simulink model "week8_heading_control"  (R2026a)
settings: Solver=VariableStepAuto
values from neighbouring files (symbols this model uses):
  alpha = (1 - sind(phi_lead))/(1 + sind(phi_lead))    [Week8.m]
  B = 0.15    [Week8.m]
  D = 3.2e-7    (= 3.2e-07)    [Week8.m]
  gear = 9.6    [Week8.m]
  J_new = 5.4836e-6    (= 5.4836e-06)    [Week8.m]
  Kb = 0.009    [Week8.m]
  Kp_P = 0.05    [Week8.m]
  Kph = sqrt(alpha)/mag(k_wc)    [Week8.m]
  Kt = 0.009    [Week8.m]
  L = 0.01    [Week8.m]
  R = 6.8    [Week8.m]
  taud = 1/(wc_lead*sqrt(alpha))    [Week8.m]
  Ts = 0.001    [Week8.m]
  useZOH = 1    [Week8.m]
  wrad = 0.0315    [Week8.m]
libraries: simulink x1
settings Model: Creator=sophiewinther  LastModifiedBy=sahra

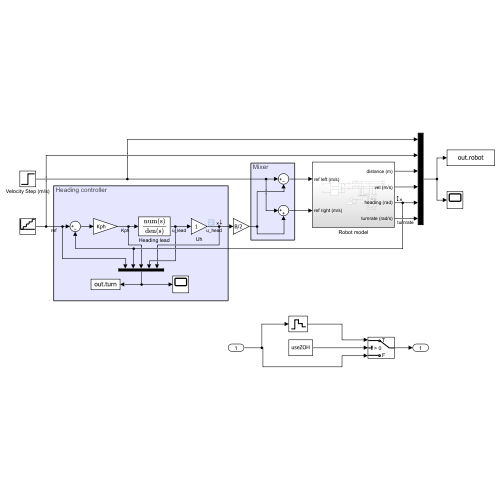
[thumbnail: Simulink's stored preview of the top-level diagram]
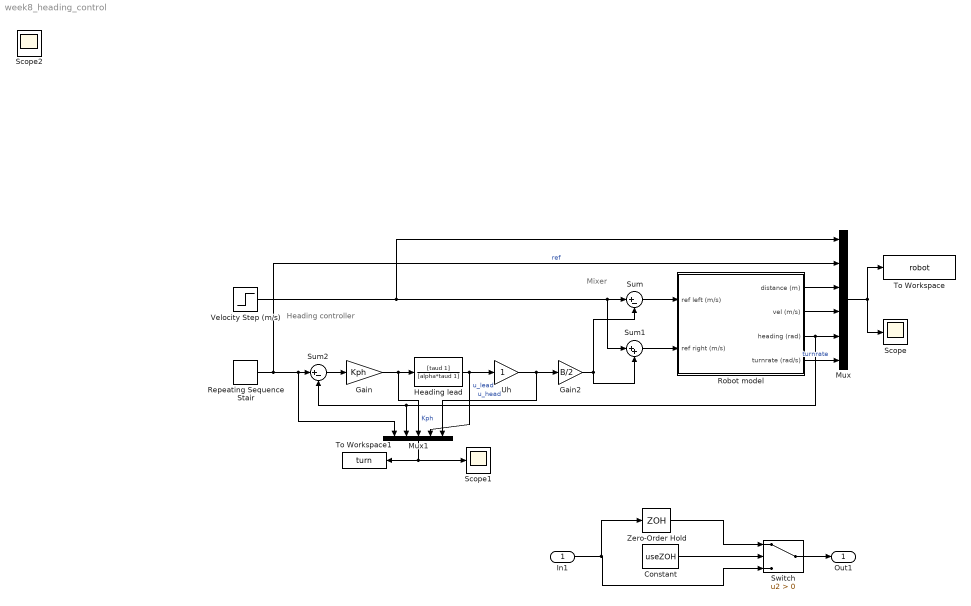
== system week8_heading_control ==
  note: Mixer
  note: Heading controller
  In1 : Inport
  Constant : Constant  Value=useZOH
  Gain : Gain  Gain=Kph
  Gain2 : Gain  Gain=B/2
  Heading lead : TransferFcn  Numerator=[taud 1]  Denominator=[alpha*taud 1]
  Mux : Mux  Inputs=6
  Mux1 : Mux  Inputs=5
  Repeating Sequence Stair : simulink/Sources/Repeating Sequence Stair  OutValues=[0 pi/2 pi 3*pi/2 2*pi ].'  tsamp=1  OutMin=[]  OutMax=[]  OutDataTypeStr=double  OutputDataTypeScalingMode=double  OutDataType=fixdt(0,8)  ConRadixGroup=Best Precision: Vector-wise  OutScaling=2^-12
  Robot model : Subsystem
  Scope : Scope
      settings: DataLoggingVariableName=ScopeData2
  Scope1 : Scope
      settings: DataLoggingVariableName=ScopeData3
  Sum : Sum  Inputs=|+-
  Sum1 : Sum  Inputs=|++
  Sum2 : Sum  Inputs=|+-
  Switch : Switch  Criteria=u2 > Threshold  SaturateOnIntegerOverflow=off  InputSameDT=off
  To Workspace : ToWorkspace  VariableName=robot  SaveFormat=Timeseries  SampleTime=-1
  To Workspace1 : ToWorkspace  VariableName=turn  SaveFormat=Timeseries  SampleTime=-1
  Uh : Gain
  Velocity Step (m/s) : Step  Time=0.1  FinalValue=0.6  SampleTime=0
  Zero-Order Hold : ZeroOrderHold  SampleTime=-1
  Out1 : Outport
  Scope2 : Scope
      settings: ActiveDisplayYMinimum=-1  ActiveDisplayYMaximum=1  DataLoggingVariableName=ScopeData4
  wires:
  Robot model/1(distance (m)) -> Mux/3
  Sum/1 -> Robot model/1(ref left (m/s))
  Repeating Sequence Stair/1 -> Mux1/1, Sum2/1, Mux/2  "ref"
  Mux/1 -> Scope/1, To Workspace/1
  Robot model/2(vel (m/s)) -> Mux/4
  Sum1/1 -> Robot model/2(ref right (m/s))
  Gain2/1 -> Sum/2, Sum1/2
  Velocity Step (m/s)/1 -> Sum/1, Sum1/1, Mux/1
  Robot model/4(turnrate (rad/s)) -> Mux/6  "turnrate"
  Robot model/3(heading (rad)) -> Mux1/2, Sum2/2, Mux/5
  Uh/1 -> Mux1/5, Gain2/1  "u_head"
  Mux1/1 -> To Workspace1/1, Scope1/1
  Sum2/1 -> Gain/1
  Gain/1 -> Mux1/3, Heading lead/1  "Kph"
  Heading lead/1 -> Mux1/4, Uh/1  "u_lead"
  Constant/1 -> Switch/2
  Zero-Order Hold/1 -> Switch/1
  In1/1 -> Zero-Order Hold/1, Switch/3
  Switch/1 -> Out1/1

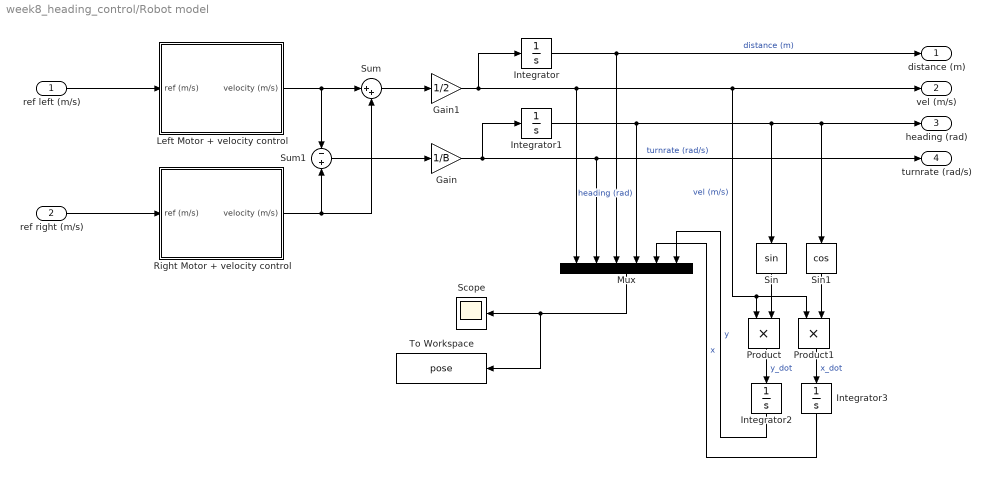
== system week8_heading_control/Robot model ==
  ref left (m/s) : Inport
  ref right (m/s) : Inport  Port=2
  Gain : Gain  Gain=1/B
  Gain1 : Gain  Gain=1/2
  Integrator{,1..3} (4 alike) : Integrator
  Left Motor + velocity control : Subsystem
  Mux : Mux  Inputs=6
  Product : Product
  Product1 : Product
  Right Motor + velocity control : Subsystem
  Scope : Scope
  Sin : Trigonometry
  Sin1 : Trigonometry  Operator=cos
  Sum : Sum  Inputs=|++
  Sum1 : Sum  Inputs=-+
  To Workspace : ToWorkspace  VariableName=pose  SaveFormat=Timeseries  SampleTime=-1
  distance (m) : Outport
  vel (m/s) : Outport  Port=2
  heading (rad) : Outport  Port=3
  turnrate (rad/s) : Outport  Port=4
  wires:
  Gain1/1 -> Integrator/1, vel (m/s)/1, Product1/1, Product/1, Mux/1  "vel (m/s)"
  Sum/1 -> Gain1/1
  Gain/1 -> Integrator1/1, turnrate (rad/s)/1, Mux/2  "turnrate (rad/s)"
  Integrator3/1 -> Mux/5  "x"
  Right Motor + velocity control/1(velocity (m/s)) -> Sum/2, Sum1/2
  Left Motor + velocity control/1(velocity (m/s)) -> Sum1/1, Sum/1
  Sum1/1 -> Gain/1
  Sin1/1 -> Product1/2
  Integrator1/1 -> Sin/1, heading (rad)/1, Sin1/1, Mux/4  "heading (rad)"
  Integrator/1 -> distance (m)/1, Mux/3  "distance (m)"
  ref left (m/s)/1 -> Left Motor + velocity control/1(ref (m/s))
  Integrator2/1 -> Mux/6  "y"
  Sin/1 -> Product/2
  ref right (m/s)/1 -> Right Motor + velocity control/1(ref (m/s))
  Mux/1 -> To Workspace/1, Scope/1
  Product1/1 -> Integrator3/1  "x_dot"
  Product/1 -> Integrator2/1  "y_dot"

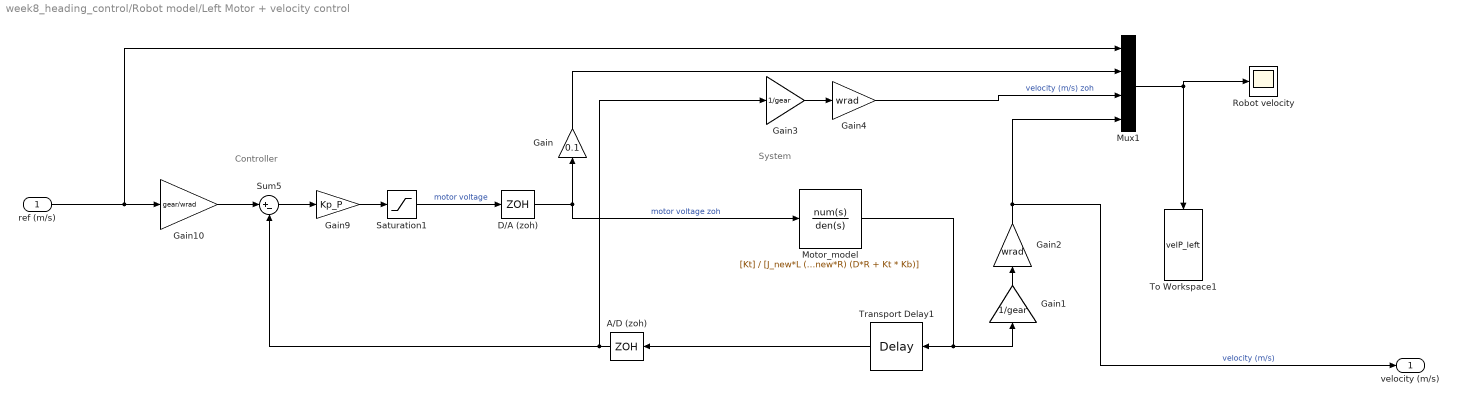
== system week8_heading_control/Robot model/Left Motor + velocity control ==
  note: Controller
  note: System
  ref (m/s) : Inport
  A/D (zoh) : ZeroOrderHold  SampleTime=Ts
  D/A (zoh) : ZeroOrderHold  SampleTime=Ts
  Gain : Gain  Gain=0.1
  Gain1 : Gain  Gain=1/gear
  Gain10 : Gain  Gain=gear/wrad
  Gain2 : Gain  Gain=wrad
  Gain3 : Gain  Gain=1/gear
  Gain4 : Gain  Gain=wrad
  Gain9 : Gain  Gain=Kp_P
  Motor_model : TransferFcn  Numerator=[Kt]  Denominator=[J_new*L (D*L + J_new*R) (D*R + Kt * Kb)]
  Mux1 : Mux
  Robot velocity : Scope
      settings: ActiveDisplayYMinimum=-60.754208750467939  ActiveDisplayYMaximum=134.00460786451399
  Saturation1 : Saturate  UpperLimit=9  LowerLimit=-9
  Sum5 : Sum  Inputs=|+-
  To Workspace1 : ToWorkspace  VariableName=velP_left  SaveFormat=Timeseries  SampleTime=-1
  Transport Delay1 : TransportDelay  DelayTime=0.01
  velocity (m/s) : Outport
  wires:
  Motor_model/1 -> Gain1/1, Transport Delay1/1
  Gain3/1 -> Gain4/1
  Gain2/1 -> velocity (m/s)/1, Mux1/4  "velocity (m/s)"
  Mux1/1 -> Robot velocity/1, To Workspace1/1
  Transport Delay1/1 -> A/D (zoh)/1
  Sum5/1 -> Gain9/1
  Gain10/1 -> Sum5/1
  A/D (zoh)/1 -> Sum5/2, Gain3/1
  Saturation1/1 -> D/A (zoh)/1  "motor voltage"
  Gain/1 -> Mux1/2
  Gain1/1 -> Gain2/1
  Gain9/1 -> Saturation1/1
  ref (m/s)/1 -> Gain10/1, Mux1/1
  D/A (zoh)/1 -> Motor_model/1, Gain/1  "motor voltage zoh"
  Gain4/1 -> Mux1/3  "velocity (m/s) zoh"

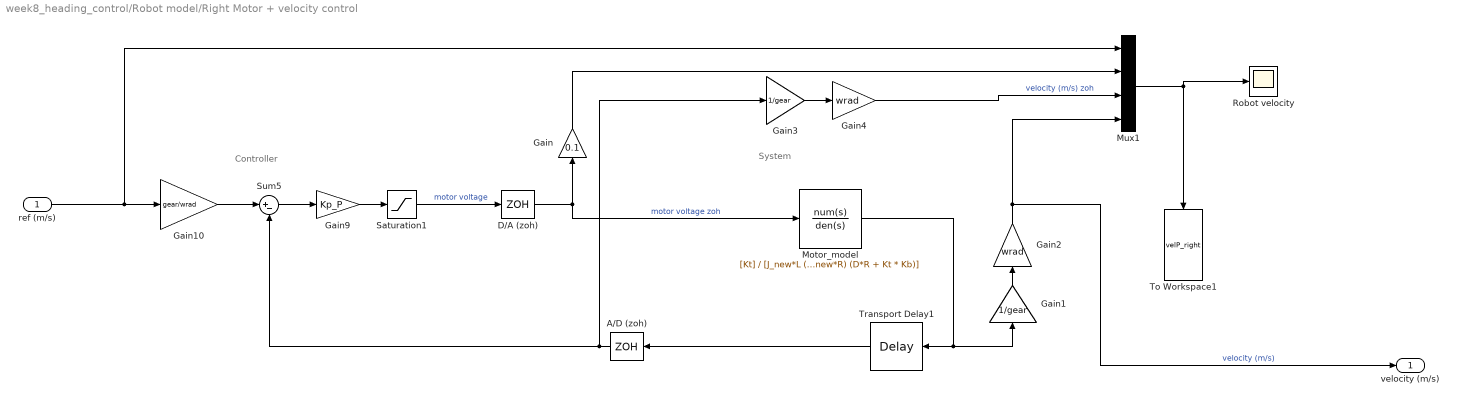
== system week8_heading_control/Robot model/Right Motor + velocity control ==
  note: Controller
  note: System
  ref (m/s) : Inport
  A/D (zoh) : ZeroOrderHold  SampleTime=Ts
  D/A (zoh) : ZeroOrderHold  SampleTime=Ts
  Gain : Gain  Gain=0.1
  Gain1 : Gain  Gain=1/gear
  Gain10 : Gain  Gain=gear/wrad
  Gain2 : Gain  Gain=wrad
  Gain3 : Gain  Gain=1/gear
  Gain4 : Gain  Gain=wrad
  Gain9 : Gain  Gain=Kp_P
  Motor_model : TransferFcn  Numerator=[Kt]  Denominator=[J_new*L (D*L + J_new*R) (D*R + Kt * Kb)]
  Mux1 : Mux
  Robot velocity : Scope
      settings: ActiveDisplayYMinimum=-60.754208750467939  ActiveDisplayYMaximum=134.00460786451399
  Saturation1 : Saturate  UpperLimit=9  LowerLimit=-9
  Sum5 : Sum  Inputs=|+-
  To Workspace1 : ToWorkspace  VariableName=velP_right  SaveFormat=Timeseries  SampleTime=-1
  Transport Delay1 : TransportDelay  DelayTime=0.01
  velocity (m/s) : Outport
  wires:
  Motor_model/1 -> Gain1/1, Transport Delay1/1
  Gain3/1 -> Gain4/1
  Gain2/1 -> velocity (m/s)/1, Mux1/4  "velocity (m/s)"
  Mux1/1 -> Robot velocity/1, To Workspace1/1
  Transport Delay1/1 -> A/D (zoh)/1
  Sum5/1 -> Gain9/1
  Gain10/1 -> Sum5/1
  A/D (zoh)/1 -> Sum5/2, Gain3/1
  Saturation1/1 -> D/A (zoh)/1  "motor voltage"
  Gain/1 -> Mux1/2
  Gain1/1 -> Gain2/1
  Gain9/1 -> Saturation1/1
  ref (m/s)/1 -> Gain10/1, Mux1/1
  D/A (zoh)/1 -> Motor_model/1, Gain/1  "motor voltage zoh"
  Gain4/1 -> Mux1/3  "velocity (m/s) zoh"
